simulink model "all_afc_0001_0365"  (R2026a)
settings: Solver=ode15s  StopTime=simTime  FixedStep=5e-05  RelTol=1e-06  AbsTol=1e-06
undefined symbols (not defined in the file): AF_sensor_tol, fault_time, fuel_inj_tol, MAF_sensor_tol, measureTime, simTime, spec_num
(part 2 of 3)

== system all_afc_0001_0365/Model 1/Cylinder and Exhaust/A//F_sensor ==
  In : Inport
  A/F_sensor : Gain  OutDataTypeStr=double
  FIMWB_133 : Subsystem  Tag=fimwb.fault.133
  FIMWB_134 : Subsystem  Tag=fimwb.fault.134
  FIMWB_135 : Subsystem  Tag=fimwb.fault.135
  Filter : Subsystem
  Out : Outport  VectorParamsAs1DForOutWhenUnconnected=off
  wires:
  In/1 -> FIMWB_133/1(Original)
  FIMWB_133/1(Result) -> Filter/1(In)
  A/F_sensor/1 -> FIMWB_134/1(Original)
  FIMWB_134/1(Result) -> Out/1
  Filter/1(Out) -> FIMWB_135/1(Original)
  FIMWB_135/1(Result) -> A/F_sensor/1

== system all_afc_0001_0365/Model 1/Cylinder and Exhaust/FIMWB_125 ==
  Original : Inport
  Result : Outport
  wires:
  Original/1 -> Result/1

== system all_afc_0001_0365/Model 1/Cylinder and Exhaust/FIMWB_126 ==
  Original : Inport
  Result : Outport
  wires:
  Original/1 -> Result/1

== system all_afc_0001_0365/Model 1/Cylinder and Exhaust/FIMWB_127 ==
  Original : Inport
  Result : Outport
  wires:
  Original/1 -> Result/1

== system all_afc_0001_0365/Model 1/Cylinder and Exhaust/FIMWB_128 ==
  Original : Inport
  Result : Outport
  wires:
  Original/1 -> Result/1

== system all_afc_0001_0365/Model 1/Cylinder and Exhaust/FIMWB_129 ==
  Original : Inport
  Result : Outport
  wires:
  Original/1 -> Result/1

== system all_afc_0001_0365/Model 1/Cylinder and Exhaust/FIMWB_130 ==
  Original : Inport
  Result : Outport
  wires:
  Original/1 -> Result/1

== system all_afc_0001_0365/Model 1/Cylinder and Exhaust/FIMWB_131 ==
  Original : Inport
  Result : Outport
  wires:
  Original/1 -> Result/1

== system all_afc_0001_0365/Model 1/Cylinder and Exhaust/FIMWB_132 ==
  Original : Inport
  Result : Outport
  wires:
  Original/1 -> Result/1

== system all_afc_0001_0365/Model 1/Cylinder and Exhaust/FIMWB_141 ==
  Original : Inport
  Result : Outport
  wires:
  Original/1 -> Result/1

== system all_afc_0001_0365/Model 1/Cylinder and Exhaust/FIMWB_142 ==
  Original : Inport
  Result : Outport
  wires:
  Original/1 -> Result/1

== system all_afc_0001_0365/Model 1/Cylinder and Exhaust/FIMWB_143 ==
  Original : Inport
  Result : Outport
  wires:
  Original/1 -> Result/1

== system all_afc_0001_0365/Model 1/Cylinder and Exhaust/FIMWB_149 ==
  Original : Inport
  Result : Outport
  wires:
  Original/1 -> Result/1

== system all_afc_0001_0365/Model 1/Cylinder and Exhaust/FIMWB_150 ==
  Original : Inport
  Result : Outport
  wires:
  Original/1 -> Result/1

== system all_afc_0001_0365/Model 1/Cylinder and Exhaust/FIMWB_151 ==
  Original : Inport
  Result : Outport
  wires:
  Original/1 -> Result/1

== system all_afc_0001_0365/Model 1/Cylinder and Exhaust/FIMWB_152 ==
  Original : Inport
  Result : Outport
  wires:
  Original/1 -> Result/1

== system all_afc_0001_0365/Model 1/Cylinder and Exhaust/FIMWB_153 ==
  Original : Inport
  Result : Outport
  wires:
  Original/1 -> Result/1

== system all_afc_0001_0365/Model 1/Cylinder and Exhaust/FIMWB_154 ==
  Original : Inport
  Result : Outport
  wires:
  Original/1 -> Result/1

== system all_afc_0001_0365/Model 1/Cylinder and Exhaust/FIMWB_155 ==
  Original : Inport
  Result : Outport
  wires:
  Original/1 -> Result/1

== system all_afc_0001_0365/Model 1/Cylinder and Exhaust/FIMWB_156 ==
  Original : Inport
  Result : Outport
  wires:
  Original/1 -> Result/1

== system all_afc_0001_0365/Model 1/Cylinder and Exhaust/FIMWB_157 ==
  Original : Inport
  Result : Outport
  wires:
  Original/1 -> Result/1

== system all_afc_0001_0365/Model 1/Cylinder and Exhaust/FIMWB_304 ==
  Original : Inport
  Operand1 : Inport  Port=2
  Operand2 : Inport  Port=3
  Unused2 : Terminator
  Unused3 : Terminator
  Result : Outport
  wires:
  Original/1 -> Result/1
  Operand1/1 -> Unused2/1
  Operand2/1 -> Unused3/1

== system all_afc_0001_0365/Model 1/Cylinder and Exhaust/FIMWB_306 ==
  Original : Inport
  Operand1 : Inport  Port=2
  Operand2 : Inport  Port=3
  Unused2 : Terminator
  Unused3 : Terminator
  Result : Outport
  wires:
  Original/1 -> Result/1
  Operand1/1 -> Unused2/1
  Operand2/1 -> Unused3/1

== system all_afc_0001_0365/Model 1/Cylinder and Exhaust/FIMWB_342 ==
  Original : Inport
  Result : Outport
  wires:
  Original/1 -> Result/1

== system all_afc_0001_0365/Model 1/Cylinder and Exhaust/FIMWB_343 ==
  Original : Inport
  Result : Outport
  wires:
  Original/1 -> Result/1

== system all_afc_0001_0365/Model 1/Cylinder and Exhaust/FIMWB_344 ==
  Original : Inport
  Result : Outport
  wires:
  Original/1 -> Result/1

== system all_afc_0001_0365/Model 1/Cylinder and Exhaust/FIMWB_347 ==
  Original : Inport
  Result : Outport
  wires:
  Original/1 -> Result/1

== system all_afc_0001_0365/Model 1/Cylinder and Exhaust/Filter ==
  in : Inport
  FIMWB_144 : Subsystem  Tag=fimwb.fault.144
  FIMWB_145 : Subsystem  Tag=fimwb.fault.145
  FIMWB_146 : Subsystem  Tag=fimwb.fault.146
  FIMWB_147 : Subsystem  Tag=fimwb.fault.147
  FIMWB_148 : Subsystem  Tag=fimwb.fault.148
  FIMWB_305 : Subsystem  Tag=fimwb.fault.305
  FIMWB_346 : Subsystem  Tag=fimwb.fault.346
  Gain1 : Gain  Gain=10
  Integrator : Integrator  InitialCondition=14.7
  Sum : Sum  Inputs=|+-
  out : Outport  VectorParamsAs1DForOutWhenUnconnected=off
  wires:
  Sum/1 -> FIMWB_305/1(Original)
  Integrator/1 -> FIMWB_346/1(Original)
  FIMWB_346/1(Result) -> FIMWB_146/1(Original), FIMWB_147/1(Original)
  in/1 -> FIMWB_144/1(Original)
  FIMWB_144/1(Result) -> Sum/1, FIMWB_305/2(Operand1)
  Gain1/1 -> FIMWB_145/1(Original)
  FIMWB_145/1(Result) -> Integrator/1
  FIMWB_146/1(Result) -> Sum/2, FIMWB_305/3(Operand2)
  FIMWB_147/1(Result) -> out/1
  FIMWB_305/1(Result) -> FIMWB_148/1(Original)
  FIMWB_148/1(Result) -> Gain1/1

== system all_afc_0001_0365/Model 1/Intake Manifold/FIMWB_174 ==
  Original : Inport
  Result : Outport
  wires:
  Original/1 -> Result/1

== system all_afc_0001_0365/Model 1/Intake Manifold/FIMWB_175 ==
  Original : Inport
  Result : Outport
  wires:
  Original/1 -> Result/1

== system all_afc_0001_0365/Model 1/Intake Manifold/FIMWB_176 ==
  Original : Inport
  Result : Outport
  wires:
  Original/1 -> Result/1

== system all_afc_0001_0365/Model 1/Intake Manifold/FIMWB_177 ==
  Original : Inport
  Result : Outport
  wires:
  Original/1 -> Result/1

== system all_afc_0001_0365/Model 1/Intake Manifold/FIMWB_178 ==
  Original : Inport
  Result : Outport
  wires:
  Original/1 -> Result/1

== system all_afc_0001_0365/Model 1/Intake Manifold/FIMWB_179 ==
  Original : Inport
  Result : Outport
  wires:
  Original/1 -> Result/1

== system all_afc_0001_0365/Model 1/Intake Manifold/FIMWB_180 ==
  Original : Inport
  Result : Outport
  wires:
  Original/1 -> Result/1

== system all_afc_0001_0365/Model 1/Intake Manifold/FIMWB_181 ==
  Original : Inport
  Result : Outport
  wires:
  Original/1 -> Result/1

== system all_afc_0001_0365/Model 1/Intake Manifold/FIMWB_182 ==
  Original : Inport
  Result : Outport
  wires:
  Original/1 -> Result/1

== system all_afc_0001_0365/Model 1/Intake Manifold/FIMWB_183 ==
  Original : Inport
  Result : Outport
  wires:
  Original/1 -> Result/1

== system all_afc_0001_0365/Model 1/Intake Manifold/FIMWB_307 ==
  Original : Inport
  Operand1 : Inport  Port=2
  Operand2 : Inport  Port=3
  Unused2 : Terminator
  Unused3 : Terminator
  Result : Outport
  wires:
  Original/1 -> Result/1
  Operand1/1 -> Unused2/1
  Operand2/1 -> Unused3/1

== system all_afc_0001_0365/Model 1/Intake Manifold/FIMWB_348 ==
  Original : Inport
  Result : Outport
  wires:
  Original/1 -> Result/1

== system all_afc_0001_0365/Model 1/Intake Manifold/FIMWB_349 ==
  Original : Inport
  Result : Outport
  wires:
  Original/1 -> Result/1

== system all_afc_0001_0365/Model 1/Throttle/FIMWB_188 ==
  Original : Inport
  Result : Outport
  wires:
  Original/1 -> Result/1

== system all_afc_0001_0365/Model 1/Throttle/FIMWB_189 ==
  Original : Inport
  Result : Outport
  wires:
  Original/1 -> Result/1

== system all_afc_0001_0365/Model 1/Throttle/FIMWB_190 ==
  Original : Inport
  Result : Outport
  wires:
  Original/1 -> Result/1

== system all_afc_0001_0365/Model 1/Throttle/FIMWB_191 ==
  Original : Inport
  Result : Outport
  wires:
  Original/1 -> Result/1

== system all_afc_0001_0365/Model 1/Throttle/FIMWB_192 ==
  Original : Inport
  Result : Outport
  wires:
  Original/1 -> Result/1

== system all_afc_0001_0365/Model 1/Throttle/FIMWB_193 ==
  Original : Inport
  Result : Outport
  wires:
  Original/1 -> Result/1

== system all_afc_0001_0365/Model 1/Throttle/FIMWB_194 ==
  Original : Inport
  Result : Outport
  wires:
  Original/1 -> Result/1

== system all_afc_0001_0365/Model 1/Throttle/FIMWB_195 ==
  Original : Inport
  Result : Outport
  wires:
  Original/1 -> Result/1

== system all_afc_0001_0365/Model 1/Throttle/FIMWB_196 ==
  Original : Inport
  Result : Outport
  wires:
  Original/1 -> Result/1

== system all_afc_0001_0365/Model 1/Throttle/FIMWB_197 ==
  Original : Inport
  Result : Outport
  wires:
  Original/1 -> Result/1

== system all_afc_0001_0365/Model 1/Throttle/FIMWB_198 ==
  Original : Inport
  Result : Outport
  wires:
  Original/1 -> Result/1

== system all_afc_0001_0365/Model 1/Throttle/FIMWB_199 ==
  Original : Inport
  Result : Outport
  wires:
  Original/1 -> Result/1

== system all_afc_0001_0365/Model 1/Throttle/FIMWB_200 ==
  Original : Inport
  Result : Outport
  wires:
  Original/1 -> Result/1

== system all_afc_0001_0365/Model 1/Throttle/FIMWB_201 ==
  Original : Inport
  Result : Outport
  wires:
  Original/1 -> Result/1

== system all_afc_0001_0365/Model 1/Throttle/FIMWB_202 ==
  Original : Inport
  Result : Outport
  wires:
  Original/1 -> Result/1

== system all_afc_0001_0365/Model 1/Throttle/FIMWB_203 ==
  Original : Inport
  Result : Outport
  wires:
  Original/1 -> Result/1

== system all_afc_0001_0365/Model 1/Throttle/FIMWB_204 ==
  Original : Inport
  Result : Outport
  wires:
  Original/1 -> Result/1

== system all_afc_0001_0365/Model 1/Throttle/FIMWB_205 ==
  Original : Inport
  Result : Outport
  wires:
  Original/1 -> Result/1

== system all_afc_0001_0365/Model 1/Throttle/FIMWB_309 ==
  Original : Inport
  Operand1 : Inport  Port=2
  Operand2 : Inport  Port=3
  Operand3 : Inport  Port=4
  Unused2 : Terminator
  Unused3 : Terminator
  Unused4 : Terminator
  Result : Outport
  wires:
  Original/1 -> Result/1
  Operand1/1 -> Unused2/1
  Operand2/1 -> Unused3/1
  Operand3/1 -> Unused4/1

== system all_afc_0001_0365/Model 1/Throttle/FIMWB_310 ==
  Original : Inport
  Operand1 : Inport  Port=2
  Operand2 : Inport  Port=3
  Unused2 : Terminator
  Unused3 : Terminator
  Result : Outport
  wires:
  Original/1 -> Result/1
  Operand1/1 -> Unused2/1
  Operand2/1 -> Unused3/1

== system all_afc_0001_0365/Model 1/Throttle/FIMWB_311 ==
  Original : Inport
  Operand1 : Inport  Port=2
  Operand2 : Inport  Port=3
  Unused2 : Terminator
  Unused3 : Terminator
  Result : Outport
  wires:
  Original/1 -> Result/1
  Operand1/1 -> Unused2/1
  Operand2/1 -> Unused3/1

== system all_afc_0001_0365/Model 1/Throttle/FIMWB_312 ==
  Original : Inport
  Operand1 : Inport  Port=2
  Operand2 : Inport  Port=3
  Unused2 : Terminator
  Unused3 : Terminator
  Result : Outport
  wires:
  Original/1 -> Result/1
  Operand1/1 -> Unused2/1
  Operand2/1 -> Unused3/1

== system all_afc_0001_0365/Model 1/Throttle/FIMWB_351 ==
  Original : Inport
  Result : Outport
  wires:
  Original/1 -> Result/1

== system all_afc_0001_0365/Model 1/Throttle/FIMWB_352 ==
  Original : Inport
  Result : Outport
  wires:
  Original/1 -> Result/1

== system all_afc_0001_0365/Model 1/Throttle/FIMWB_353 ==
  Original : Inport
  Result : Outport
  wires:
  Original/1 -> Result/1

== system all_afc_0001_0365/Model 1/Wall wetting/FIMWB_208 ==
  Original : Inport
  Result : Outport
  wires:
  Original/1 -> Result/1

== system all_afc_0001_0365/Model 1/Wall wetting/FIMWB_209 ==
  Original : Inport
  Result : Outport
  wires:
  Original/1 -> Result/1

== system all_afc_0001_0365/Model 1/Wall wetting/FIMWB_210 ==
  Original : Inport
  Result : Outport
  wires:
  Original/1 -> Result/1

== system all_afc_0001_0365/Model 1/Wall wetting/FIMWB_211 ==
  Original : Inport
  Result : Outport
  wires:
  Original/1 -> Result/1

== system all_afc_0001_0365/Model 1/Wall wetting/FIMWB_212 ==
  Original : Inport
  Result : Outport
  wires:
  Original/1 -> Result/1

== system all_afc_0001_0365/Model 1/Wall wetting/FIMWB_213 ==
  Original : Inport
  Result : Outport
  wires:
  Original/1 -> Result/1

== system all_afc_0001_0365/Model 1/Wall wetting/FIMWB_214 ==
  Original : Inport
  Result : Outport
  wires:
  Original/1 -> Result/1

== system all_afc_0001_0365/Model 1/Wall wetting/FIMWB_215 ==
  Original : Inport
  Result : Outport
  wires:
  Original/1 -> Result/1

== system all_afc_0001_0365/Model 1/Wall wetting/FIMWB_216 ==
  Original : Inport
  Result : Outport
  wires:
  Original/1 -> Result/1

== system all_afc_0001_0365/Model 1/Wall wetting/FIMWB_217 ==
  Original : Inport
  Result : Outport
  wires:
  Original/1 -> Result/1

== system all_afc_0001_0365/Model 1/Wall wetting/FIMWB_218 ==
  Original : Inport
  Result : Outport
  wires:
  Original/1 -> Result/1

== system all_afc_0001_0365/Model 1/Wall wetting/FIMWB_219 ==
  Original : Inport
  Result : Outport
  wires:
  Original/1 -> Result/1

== system all_afc_0001_0365/Model 1/Wall wetting/FIMWB_220 ==
  Original : Inport
  Result : Outport
  wires:
  Original/1 -> Result/1

== system all_afc_0001_0365/Model 1/Wall wetting/FIMWB_221 ==
  Original : Inport
  Result : Outport
  wires:
  Original/1 -> Result/1

== system all_afc_0001_0365/Model 1/Wall wetting/FIMWB_222 ==
  Original : Inport
  Result : Outport
  wires:
  Original/1 -> Result/1

== system all_afc_0001_0365/Model 1/Wall wetting/FIMWB_223 ==
  Original : Inport
  Result : Outport
  wires:
  Original/1 -> Result/1

== system all_afc_0001_0365/Model 1/Wall wetting/FIMWB_224 ==
  Original : Inport
  Result : Outport
  wires:
  Original/1 -> Result/1

== system all_afc_0001_0365/Model 1/Wall wetting/FIMWB_225 ==
  Original : Inport
  Result : Outport
  wires:
  Original/1 -> Result/1

== system all_afc_0001_0365/Model 1/Wall wetting/FIMWB_226 ==
  Original : Inport
  Result : Outport
  wires:
  Original/1 -> Result/1

== system all_afc_0001_0365/Model 1/Wall wetting/FIMWB_227 ==
  Original : Inport
  Result : Outport
  wires:
  Original/1 -> Result/1

== system all_afc_0001_0365/Model 1/Wall wetting/FIMWB_228 ==
  Original : Inport
  Result : Outport
  wires:
  Original/1 -> Result/1

== system all_afc_0001_0365/Model 1/Wall wetting/FIMWB_229 ==
  Original : Inport
  Result : Outport
  wires:
  Original/1 -> Result/1

== system all_afc_0001_0365/Model 1/Wall wetting/FIMWB_230 ==
  Original : Inport
  Result : Outport
  wires:
  Original/1 -> Result/1

== system all_afc_0001_0365/Model 1/Wall wetting/FIMWB_231 ==
  Original : Inport
  Result : Outport
  wires:
  Original/1 -> Result/1

== system all_afc_0001_0365/Model 1/Wall wetting/FIMWB_313 ==
  Original : Inport
  Operand1 : Inport  Port=2
  Operand2 : Inport  Port=3
  Unused2 : Terminator
  Unused3 : Terminator
  Result : Outport
  wires:
  Original/1 -> Result/1
  Operand1/1 -> Unused2/1
  Operand2/1 -> Unused3/1

== system all_afc_0001_0365/Model 1/Wall wetting/FIMWB_314 ==
  Original : Inport
  Operand1 : Inport  Port=2
  Operand2 : Inport  Port=3
  Unused2 : Terminator
  Unused3 : Terminator
  Result : Outport
  wires:
  Original/1 -> Result/1
  Operand1/1 -> Unused2/1
  Operand2/1 -> Unused3/1

== system all_afc_0001_0365/Model 1/Wall wetting/FIMWB_315 ==
  Original : Inport
  Operand1 : Inport  Port=2
  Operand2 : Inport  Port=3
  Unused2 : Terminator
  Unused3 : Terminator
  Result : Outport
  wires:
  Original/1 -> Result/1
  Operand1/1 -> Unused2/1
  Operand2/1 -> Unused3/1

== system all_afc_0001_0365/Model 1/Wall wetting/FIMWB_316 ==
  Original : Inport
  Operand1 : Inport  Port=2
  Operand2 : Inport  Port=3
  Unused2 : Terminator
  Unused3 : Terminator
  Result : Outport
  wires:
  Original/1 -> Result/1
  Operand1/1 -> Unused2/1
  Operand2/1 -> Unused3/1

== system all_afc_0001_0365/Model 1/Wall wetting/FIMWB_317 ==
  Original : Inport
  Operand1 : Inport  Port=2
  Operand2 : Inport  Port=3
  Unused2 : Terminator
  Unused3 : Terminator
  Result : Outport
  wires:
  Original/1 -> Result/1
  Operand1/1 -> Unused2/1
  Operand2/1 -> Unused3/1

== system all_afc_0001_0365/Model 1/Wall wetting/FIMWB_318 ==
  Original : Inport
  Operand1 : Inport  Port=2
  Operand2 : Inport  Port=3
  Unused2 : Terminator
  Unused3 : Terminator
  Result : Outport
  wires:
  Original/1 -> Result/1
  Operand1/1 -> Unused2/1
  Operand2/1 -> Unused3/1

== system all_afc_0001_0365/Model 1/Wall wetting/FIMWB_354 ==
  Original : Inport
  Result : Outport
  wires:
  Original/1 -> Result/1

== system all_afc_0001_0365/Model 1/Wall wetting/FIMWB_355 ==
  Original : Inport
  Result : Outport
  wires:
  Original/1 -> Result/1

== system all_afc_0001_0365/Model 1/Wall wetting/FIMWB_356 ==
  Original : Inport
  Result : Outport
  wires:
  Original/1 -> Result/1

== system all_afc_0001_0365/Model 1/Wall wetting/FIMWB_357 ==
  Original : Inport
  Result : Outport
  wires:
  Original/1 -> Result/1

== system all_afc_0001_0365/Model 1/Wall wetting/FIMWB_358 ==
  Original : Inport
  Result : Outport
  wires:
  Original/1 -> Result/1

== system all_afc_0001_0365/V&V stub system/Calcuate Error/FIMWB_241 ==
  Original : Inport
  Result : Outport
  wires:
  Original/1 -> Result/1

== system all_afc_0001_0365/V&V stub system/Calcuate Error/FIMWB_242 ==
  Original : Inport
  Result : Outport
  wires:
  Original/1 -> Result/1

== system all_afc_0001_0365/V&V stub system/Calcuate Error/FIMWB_243 ==
  Original : Inport
  Result : Outport
  wires:
  Original/1 -> Result/1

== system all_afc_0001_0365/V&V stub system/Calcuate Error/FIMWB_244 ==
  Original : Inport
  Result : Outport
  wires:
  Original/1 -> Result/1

== system all_afc_0001_0365/V&V stub system/Calcuate Error/FIMWB_245 ==
  Original : Inport
  Result : Outport
  wires:
  Original/1 -> Result/1

== system all_afc_0001_0365/V&V stub system/Calcuate Error/FIMWB_246 ==
  Original : Inport
  Result : Outport
  wires:
  Original/1 -> Result/1

== system all_afc_0001_0365/V&V stub system/Calcuate Error/FIMWB_247 ==
  Original : Inport
  Result : Outport
  wires:
  Original/1 -> Result/1

== system all_afc_0001_0365/V&V stub system/Calcuate Error/FIMWB_255 ==
  Original : Inport
  Result : Outport
  wires:
  Original/1 -> Result/1

== system all_afc_0001_0365/V&V stub system/Calcuate Error/FIMWB_272 ==
  Original : Inport
  Result : Outport
  wires:
  Original/1 -> Result/1

== system all_afc_0001_0365/V&V stub system/Calcuate Error/FIMWB_273 ==
  Original : Inport
  Result : Outport
  wires:
  Original/1 -> Result/1

== system all_afc_0001_0365/V&V stub system/Calcuate Error/FIMWB_274 ==
  Original : Inport
  Result : Outport
  wires:
  Original/1 -> Result/1

== system all_afc_0001_0365/V&V stub system/Calcuate Error/FIMWB_362 ==
  Original : Inport
  Result : Outport
  wires:
  Original/1 -> Result/1

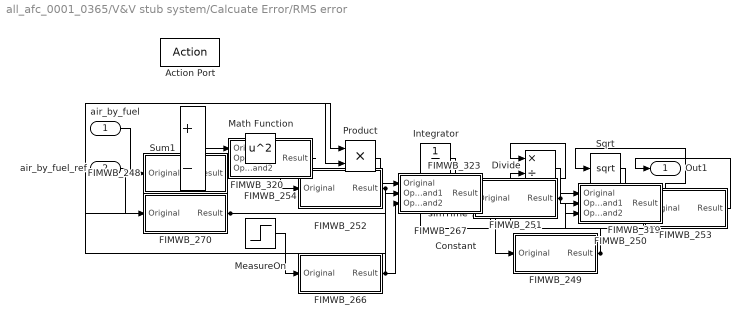
== system all_afc_0001_0365/V&V stub system/Calcuate Error/RMS error ==
  "air_by_fuel " : Inport
  air_by_fuel_ref : Inport  Port=2
  Action Port : ActionPort  ActionPortLabel=case: { }
  Constant : Constant  Value=simTime-10
  Divide : Product  Inputs=*/
  FIMWB_248 : Subsystem  Tag=fimwb.fault.248
  FIMWB_249 : Subsystem  Tag=fimwb.fault.249
  FIMWB_250 : Subsystem  Tag=fimwb.fault.250
  FIMWB_251 : Subsystem  Tag=fimwb.fault.251
  FIMWB_252 : Subsystem  Tag=fimwb.fault.252
  FIMWB_253 : Subsystem  Tag=fimwb.fault.253
  FIMWB_254 : Subsystem  Tag=fimwb.fault.254
  FIMWB_266 : Subsystem  Tag=fimwb.fault.266
  FIMWB_267 : Subsystem  Tag=fimwb.fault.267
  FIMWB_270 : Subsystem  Tag=fimwb.fault.270
  FIMWB_319 : Subsystem  Tag=fimwb.fault.319
  FIMWB_320 : Subsystem  Tag=fimwb.fault.320
  FIMWB_323 : Subsystem  Tag=fimwb.fault.323
  Integrator : Integrator
  Math Function : Math  Operator=square  SignedPower=on
  MeasureOn : Step  Time=10  SampleTime=0
  Product : Product
  Sqrt : Sqrt
  Sum1 : Sum  Inputs=+-  OutDataTypeStr=Inherit: Inherit via back propagation  InputSameDT=on  RndMeth=Simplest
  Out1 : Outport  VectorParamsAs1DForOutWhenUnconnected=off
  wires:
  Divide/1 -> FIMWB_319/1(Original)
  Sum1/1 -> FIMWB_320/1(Original)
  Product/1 -> FIMWB_323/1(Original)
  "air_by_fuel "/1 -> FIMWB_248/1(Original)
  FIMWB_248/1(Result) -> Sum1/1, FIMWB_320/2(Operand1)
  Constant/1 -> FIMWB_249/1(Original)
  FIMWB_249/1(Result) -> Divide/2, FIMWB_319/3(Operand2)
  FIMWB_319/1(Result) -> FIMWB_250/1(Original)
  FIMWB_250/1(Result) -> Sqrt/1
  Integrator/1 -> FIMWB_251/1(Original)
  FIMWB_251/1(Result) -> Divide/1, FIMWB_319/2(Operand1)
  Math Function/1 -> FIMWB_252/1(Original)
  FIMWB_252/1(Result) -> Product/1, FIMWB_323/2(Operand1)
  Sqrt/1 -> FIMWB_253/1(Original)
  FIMWB_253/1(Result) -> Out1/1
  FIMWB_320/1(Result) -> FIMWB_254/1(Original)
  FIMWB_254/1(Result) -> Math Function/1
  MeasureOn/1 -> FIMWB_266/1(Original)
  FIMWB_266/1(Result) -> Product/2, FIMWB_323/3(Operand2)
  FIMWB_323/1(Result) -> FIMWB_267/1(Original)
  FIMWB_267/1(Result) -> Integrator/1
  air_by_fuel_ref/1 -> FIMWB_270/1(Original)
  FIMWB_270/1(Result) -> Sum1/2, FIMWB_320/3(Operand2)

== system all_afc_0001_0365/V&V stub system/Calcuate Error/over(under)shoot ==
  "air_by_fuel " : Inport
  air_by_fuel_ref : Inport  Port=2
  Action Port : ActionPort  ActionPortLabel=case: { }
  Constant : Constant
  Divide : Product  Inputs=*/
  FIMWB_256 : Subsystem  Tag=fimwb.fault.256
  FIMWB_257 : Subsystem  Tag=fimwb.fault.257
  FIMWB_258 : Subsystem  Tag=fimwb.fault.258
  FIMWB_259 : Subsystem  Tag=fimwb.fault.259
  FIMWB_271 : Subsystem  Tag=fimwb.fault.271
  FIMWB_321 : Subsystem  Tag=fimwb.fault.321
  FIMWB_322 : Subsystem  Tag=fimwb.fault.322
  Sum1 : Sum  Inputs=+-  OutDataTypeStr=Inherit: Inherit via back propagation  InputSameDT=on  RndMeth=Simplest
  Out1 : Outport  VectorParamsAs1DForOutWhenUnconnected=off
  wires:
  Divide/1 -> FIMWB_321/1(Original)
  Sum1/1 -> FIMWB_322/1(Original)
  "air_by_fuel "/1 -> FIMWB_256/1(Original)
  FIMWB_256/1(Result) -> Divide/1, FIMWB_321/2(Operand1)
  Constant/1 -> FIMWB_257/1(Original)
  FIMWB_257/1(Result) -> Sum1/2, FIMWB_322/3(Operand2)
  FIMWB_321/1(Result) -> FIMWB_258/1(Original)
  FIMWB_258/1(Result) -> Sum1/1, FIMWB_322/2(Operand1)
  FIMWB_322/1(Result) -> FIMWB_259/1(Original)
  FIMWB_259/1(Result) -> Out1/1
  air_by_fuel_ref/1 -> FIMWB_271/1(Original)
  FIMWB_271/1(Result) -> Divide/2, FIMWB_321/3(Operand2)

== system all_afc_0001_0365/Model 1/AF_Controller/fuel_controller/FIMWB_021 ==
  Original : Inport
  Result : Outport
  wires:
  Original/1 -> Result/1

== system all_afc_0001_0365/Model 1/AF_Controller/fuel_controller/FIMWB_022 ==
  Original : Inport
  Result : Outport
  wires:
  Original/1 -> Result/1

== system all_afc_0001_0365/Model 1/AF_Controller/fuel_controller/FIMWB_023 ==
  Original : Inport
  Result : Outport
  wires:
  Original/1 -> Result/1

== system all_afc_0001_0365/Model 1/AF_Controller/fuel_controller/FIMWB_024 ==
  Original : Inport
  Result : Outport
  wires:
  Original/1 -> Result/1

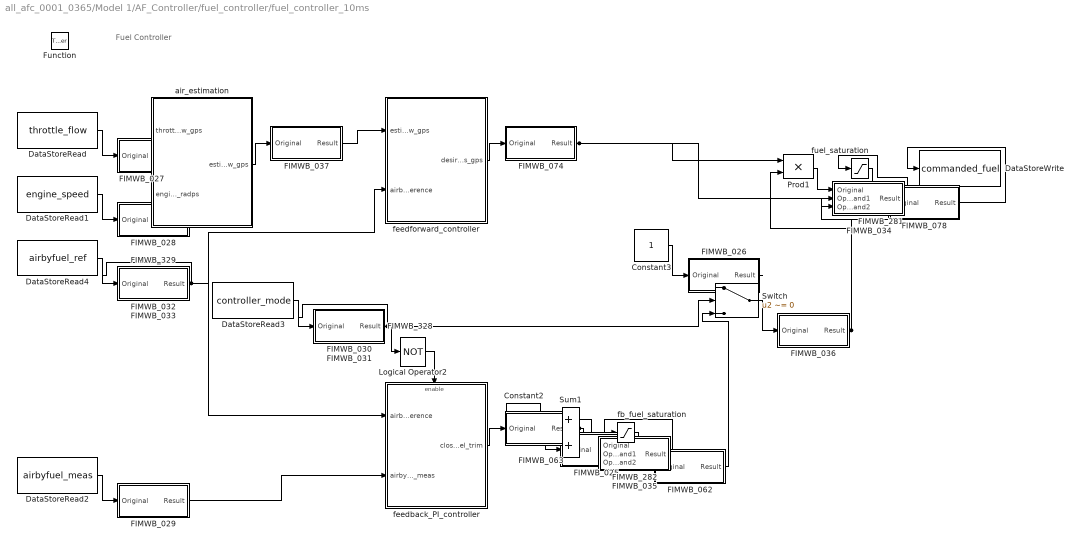
== system all_afc_0001_0365/Model 1/AF_Controller/fuel_controller/fuel_controller_10ms ==
  note: Fuel Controller
  Function : TriggerPort  VariantControl=(inherit)
  Constant2 : Constant  OutDataTypeStr=single
  Constant3 : Constant  OutDataTypeStr=single
  DataStoreRead : DataStoreRead  DataStoreName=throttle_flow  IndexOptions=Index vector (dialog)  Indices=1  OutputSizes=1
  DataStoreRead1 : DataStoreRead  DataStoreName=engine_speed  IndexOptions=Index vector (dialog)  Indices=1  OutputSizes=1
  DataStoreRead2 : DataStoreRead  DataStoreName=airbyfuel_meas  IndexOptions=Index vector (dialog)  Indices=1  OutputSizes=1
  DataStoreRead3 : DataStoreRead  DataStoreName=controller_mode  IndexOptions=Index vector (dialog)  Indices=1  OutputSizes=1
      settings: AttributesFormatString=1: Feedforward\n0: Feedforward + Feedback
  DataStoreRead4 : DataStoreRead  DataStoreName=airbyfuel_ref  IndexOptions=Index vector (dialog)  Indices=1  OutputSizes=1
  DataStoreWrite : DataStoreWrite  DataStoreName=commanded_fuel  IndexOptions=Index vector (dialog)  Indices=1  OutputSizes=1
  FIMWB_025 : Subsystem  Tag=fimwb.fault.25
  FIMWB_026 : Subsystem  Tag=fimwb.fault.26
  FIMWB_027 : Subsystem  Tag=fimwb.fault.27
  FIMWB_028 : Subsystem  Tag=fimwb.fault.28
  FIMWB_029 : Subsystem  Tag=fimwb.fault.29
  FIMWB_030 : Subsystem  Tag=fimwb.fault.30
  FIMWB_031 : Subsystem  Tag=fimwb.fault.31
  FIMWB_032 : Subsystem  Tag=fimwb.fault.32
  FIMWB_033 : Subsystem  Tag=fimwb.fault.33
  FIMWB_034 : Subsystem  Tag=fimwb.fault.34
  FIMWB_035 : Subsystem  Tag=fimwb.fault.35
  FIMWB_036 : Subsystem  Tag=fimwb.fault.36
  FIMWB_037 : Subsystem  Tag=fimwb.fault.37
  FIMWB_062 : Subsystem  Tag=fimwb.fault.62
  FIMWB_063 : Subsystem  Tag=fimwb.fault.63
  FIMWB_074 : Subsystem  Tag=fimwb.fault.74
  FIMWB_078 : Subsystem  Tag=fimwb.fault.78
  FIMWB_281 : Subsystem  Tag=fimwb.fault.281
  FIMWB_282 : Subsystem  Tag=fimwb.fault.282
  FIMWB_328 : Subsystem  Tag=fimwb.fault.328
  FIMWB_329 : Subsystem  Tag=fimwb.fault.329
  Logical Operator2 : Logic  Operator=NOT  AllPortsSameDT=off  OutDataTypeStr=boolean
  Prod1 : Product  OutDataTypeStr=Inherit: Inherit via back propagation  RndMeth=Simplest
  Sum1 : Sum  OutDataTypeStr=Inherit: Inherit via back propagation  InputSameDT=on  RndMeth=Simplest
  Switch : Switch  Criteria=u2 ~= 0  Threshold=0.5  SaturateOnIntegerOverflow=off  InputSameDT=off
  air_estimation : Subsystem  TreatAsAtomicUnit=on
  fb_fuel_saturation : Saturate  UpperLimit=inf  LowerLimit=0  RndMeth=Round
      settings: AttributesFormatString=y >= 0
  feedback_PI_controller : Subsystem  TreatAsAtomicUnit=on
  feedforward_controller : Subsystem  TreatAsAtomicUnit=on
  fuel_saturation : Saturate  UpperLimit=1.66  LowerLimit=0.13  RndMeth=Round
      settings: AttributesFormatString=0.13 <=\ncommanded_fuel\n<= 1.66
  wires:
  Logical Operator2/1 -> feedback_PI_controller/Enable
  Prod1/1 -> FIMWB_281/1(Original)
  Sum1/1 -> FIMWB_282/1(Original)
  DataStoreRead3/1 -> FIMWB_328/1(Original)
  FIMWB_328/1(Result) -> FIMWB_030/1(Original), FIMWB_031/1(Original)
  DataStoreRead4/1 -> FIMWB_329/1(Original)
  FIMWB_329/1(Result) -> FIMWB_032/1(Original), FIMWB_033/1(Original)
  Constant2/1 -> FIMWB_025/1(Original)
  FIMWB_025/1(Result) -> Sum1/1, FIMWB_282/2(Operand1)
  Constant3/1 -> FIMWB_026/1(Original)
  FIMWB_026/1(Result) -> Switch/1
  DataStoreRead/1 -> FIMWB_027/1(Original)
  FIMWB_027/1(Result) -> air_estimation/1(throttle_flow_gps)
  DataStoreRead1/1 -> FIMWB_028/1(Original)
  FIMWB_028/1(Result) -> air_estimation/2(engine_speed_radps)
  DataStoreRead2/1 -> FIMWB_029/1(Original)
  FIMWB_029/1(Result) -> feedback_PI_controller/2(airbyfuel_meas)
  FIMWB_030/1(Result) -> Logical Operator2/1
  FIMWB_031/1(Result) -> Switch/2
  FIMWB_032/1(Result) -> feedback_PI_controller/1(airbyfuel_reference)
  FIMWB_033/1(Result) -> feedforward_controller/2(airbyfuel_reference)
  FIMWB_281/1(Result) -> FIMWB_034/1(Original)
  FIMWB_034/1(Result) -> fuel_saturation/1
  FIMWB_282/1(Result) -> FIMWB_035/1(Original)
  FIMWB_035/1(Result) -> fb_fuel_saturation/1
  Switch/1 -> FIMWB_036/1(Original)
  FIMWB_036/1(Result) -> Prod1/2, FIMWB_281/3(Operand2)
  air_estimation/1(estimated_cyl_air_flow_gps) -> FIMWB_037/1(Original)
  FIMWB_037/1(Result) -> feedforward_controller/1(estimated_cyl_air_flow_gps)
  fb_fuel_saturation/1 -> FIMWB_062/1(Original)
  FIMWB_062/1(Result) -> Switch/3
  feedback_PI_controller/1(closed_loop_fuel_trim) -> FIMWB_063/1(Original)
  FIMWB_063/1(Result) -> Sum1/2, FIMWB_282/3(Operand2)
  feedforward_controller/1(desired_fuel_mass_gps) -> FIMWB_074/1(Original)
  FIMWB_074/1(Result) -> Prod1/1, FIMWB_281/2(Operand1)
  fuel_saturation/1 -> FIMWB_078/1(Original)
  FIMWB_078/1(Result) -> DataStoreWrite/1

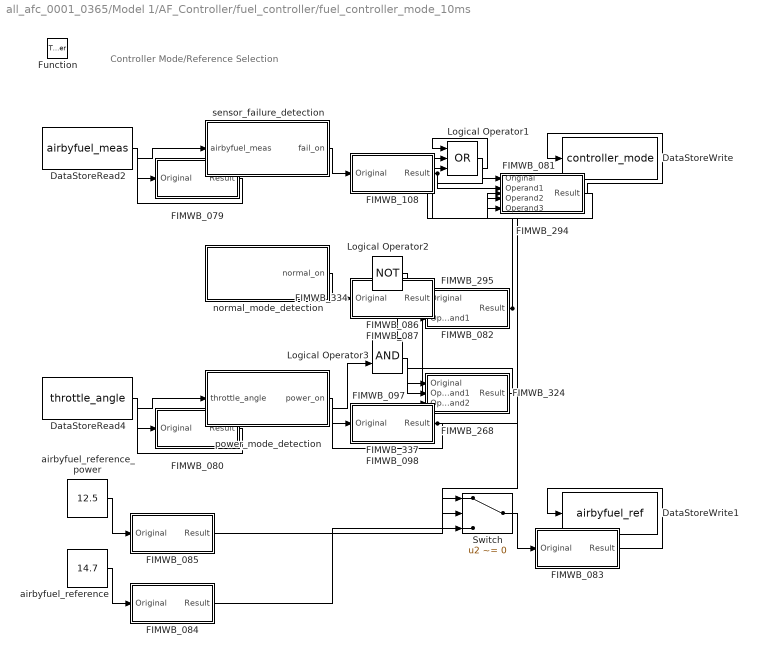
== system all_afc_0001_0365/Model 1/AF_Controller/fuel_controller/fuel_controller_mode_10ms ==
  note: Controller Mode/Reference Selection
  Function : TriggerPort  VariantControl=(inherit)
  DataStoreRead2 : DataStoreRead  DataStoreName=airbyfuel_meas  IndexOptions=Index vector (dialog)  Indices=1  OutputSizes=1
  DataStoreRead4 : DataStoreRead  DataStoreName=throttle_angle  IndexOptions=Index vector (dialog)  Indices=1  OutputSizes=1
  DataStoreWrite : DataStoreWrite  DataStoreName=controller_mode  IndexOptions=Index vector (dialog)  Indices=1  OutputSizes=1
      settings: AttributesFormatString=1: Feedforward\n0: Feedforward + Feedback
  DataStoreWrite1 : DataStoreWrite  DataStoreName=airbyfuel_ref  IndexOptions=Index vector (dialog)  Indices=1  OutputSizes=1
  FIMWB_079 : Subsystem  Tag=fimwb.fault.79
  FIMWB_080 : Subsystem  Tag=fimwb.fault.80
  FIMWB_081 : Subsystem  Tag=fimwb.fault.81
  FIMWB_082 : Subsystem  Tag=fimwb.fault.82
  FIMWB_083 : Subsystem  Tag=fimwb.fault.83
  FIMWB_084 : Subsystem  Tag=fimwb.fault.84
  FIMWB_085 : Subsystem  Tag=fimwb.fault.85
  FIMWB_086 : Subsystem  Tag=fimwb.fault.86
  FIMWB_087 : Subsystem  Tag=fimwb.fault.87
  FIMWB_097 : Subsystem  Tag=fimwb.fault.97
  FIMWB_098 : Subsystem  Tag=fimwb.fault.98
  FIMWB_108 : Subsystem  Tag=fimwb.fault.108
  FIMWB_268 : Subsystem  Tag=fimwb.fault.268
  FIMWB_294 : Subsystem  Tag=fimwb.fault.294
  FIMWB_295 : Subsystem  Tag=fimwb.fault.295
  FIMWB_324 : Subsystem  Tag=fimwb.fault.324
  FIMWB_334 : Subsystem  Tag=fimwb.fault.334
  FIMWB_337 : Subsystem  Tag=fimwb.fault.337
  Logical Operator1 : Logic  Operator=OR  Inputs=3  AllPortsSameDT=off  OutDataTypeStr=boolean
  Logical Operator2 : Logic  Operator=NOT  AllPortsSameDT=off  OutDataTypeStr=boolean
  Logical Operator3 : Logic  AllPortsSameDT=off  OutDataTypeStr=boolean
  Switch : Switch  Criteria=u2 ~= 0  SaturateOnIntegerOverflow=off  InputSameDT=off
  airbyfuel_reference : Constant  Value=14.7  OutDataTypeStr=single  SampleTime=-1
  airbyfuel_reference_power : Constant  Value=12.5  OutDataTypeStr=single  SampleTime=-1
  normal_mode_detection : Subsystem  TreatAsAtomicUnit=on
      settings: AttributesFormatString=0: Feedforward\n1: Feedforward + Feedback
  power_mode_detection : Subsystem  TreatAsAtomicUnit=on
      settings: AttributesFormatString=1: Feedforward\n0: Feedforward + Feedback
  sensor_failure_detection : Subsystem  TreatAsAtomicUnit=on
      settings: AttributesFormatString=1: Feedforward\n0: Feedforward + Feedback
  wires:
  Logical Operator1/1 -> FIMWB_294/1(Original)
  Logical Operator2/1 -> FIMWB_295/1(Original)
  Logical Operator3/1 -> FIMWB_324/1(Original)
  normal_mode_detection/1(normal_on) -> FIMWB_334/1(Original)
  FIMWB_334/1(Result) -> FIMWB_086/1(Original), FIMWB_087/1(Original)
  power_mode_detection/1(power_on) -> FIMWB_337/1(Original)
  FIMWB_337/1(Result) -> FIMWB_097/1(Original), FIMWB_098/1(Original)
  DataStoreRead2/1 -> FIMWB_079/1(Original)
  FIMWB_079/1(Result) -> sensor_failure_detection/1(airbyfuel_meas)
  DataStoreRead4/1 -> FIMWB_080/1(Original)
  FIMWB_080/1(Result) -> power_mode_detection/1(throttle_angle)
  FIMWB_294/1(Result) -> FIMWB_081/1(Original)
  FIMWB_081/1(Result) -> DataStoreWrite/1
  FIMWB_295/1(Result) -> FIMWB_082/1(Original)
  FIMWB_082/1(Result) -> Logical Operator1/2, FIMWB_294/3(Operand2)
  Switch/1 -> FIMWB_083/1(Original)
  FIMWB_083/1(Result) -> DataStoreWrite1/1
  airbyfuel_reference/1 -> FIMWB_084/1(Original)
  FIMWB_084/1(Result) -> Switch/3
  airbyfuel_reference_power/1 -> FIMWB_085/1(Original)
  FIMWB_085/1(Result) -> Switch/1
  FIMWB_086/1(Result) -> Logical Operator2/1, FIMWB_295/2(Operand1)
  FIMWB_087/1(Result) -> Logical Operator3/1, FIMWB_324/2(Operand1)
  FIMWB_097/1(Result) -> Logical Operator1/3, FIMWB_294/4(Operand3)
  FIMWB_098/1(Result) -> Logical Operator3/2, FIMWB_324/3(Operand2)
  sensor_failure_detection/1(fail_on) -> FIMWB_108/1(Original)
  FIMWB_108/1(Result) -> Logical Operator1/1, FIMWB_294/2(Operand1)
  FIMWB_324/1(Result) -> FIMWB_268/1(Original)
  FIMWB_268/1(Result) -> Switch/2

== system all_afc_0001_0365/Model 1/AF_Controller/fuel_controller/fuel_controller_pwon ==
  Function : TriggerPort  VariantControl=(inherit)
  Constant1 : Constant  OutDataTypeStr=single  SampleTime=-1
  Constant2 : Constant  Value=0.1726  OutDataTypeStr=single  SampleTime=-1
  Constant3 : Constant  Value=14.7  OutDataTypeStr=single  SampleTime=-1
  Data Type Conversion : DataTypeConversion  OutDataTypeStr=boolean  SaturateOnIntegerOverflow=off  RndMeth=Floor
  DataStoreWrite : DataStoreWrite  DataStoreName=commanded_fuel  IndexOptions=Index vector (dialog)  Indices=1  OutputSizes=1
  DataStoreWrite1 : DataStoreWrite  DataStoreName=controller_mode  IndexOptions=Index vector (dialog)  Indices=1  OutputSizes=1
  DataStoreWrite2 : DataStoreWrite  DataStoreName=airbyfuel_ref  IndexOptions=Index vector (dialog)  Indices=1  OutputSizes=1
  FIMWB_115 : Subsystem  Tag=fimwb.fault.115
  FIMWB_116 : Subsystem  Tag=fimwb.fault.116
  FIMWB_117 : Subsystem  Tag=fimwb.fault.117
  FIMWB_118 : Subsystem  Tag=fimwb.fault.118
  wires:
  Constant1/1 -> FIMWB_115/1(Original)
  FIMWB_115/1(Result) -> Data Type Conversion/1
  Constant2/1 -> FIMWB_116/1(Original)
  FIMWB_116/1(Result) -> DataStoreWrite/1
  Constant3/1 -> FIMWB_117/1(Original)
  FIMWB_117/1(Result) -> DataStoreWrite2/1
  Data Type Conversion/1 -> FIMWB_118/1(Original)
  FIMWB_118/1(Result) -> DataStoreWrite1/1

== system all_afc_0001_0365/Model 1/Cylinder and Exhaust/A//F_sensor/FIMWB_133 ==
  Original : Inport
  Result : Outport
  wires:
  Original/1 -> Result/1

== system all_afc_0001_0365/Model 1/Cylinder and Exhaust/A//F_sensor/FIMWB_134 ==
  Original : Inport
  Result : Outport
  wires:
  Original/1 -> Result/1

== system all_afc_0001_0365/Model 1/Cylinder and Exhaust/A//F_sensor/FIMWB_135 ==
  Original : Inport
  Result : Outport
  wires:
  Original/1 -> Result/1

== system all_afc_0001_0365/Model 1/Cylinder and Exhaust/A//F_sensor/Filter ==
  In : Inport
  FIMWB_136 : Subsystem  Tag=fimwb.fault.136
  FIMWB_137 : Subsystem  Tag=fimwb.fault.137
  FIMWB_138 : Subsystem  Tag=fimwb.fault.138
  FIMWB_139 : Subsystem  Tag=fimwb.fault.139
  FIMWB_140 : Subsystem  Tag=fimwb.fault.140
  FIMWB_303 : Subsystem  Tag=fimwb.fault.303
  FIMWB_345 : Subsystem  Tag=fimwb.fault.345
  Gain : Gain  Gain=50
  Integrator : Integrator  InitialCondition=14.7
  Sum : Sum  Inputs=|+-
  Out : Outport  VectorParamsAs1DForOutWhenUnconnected=off
  wires:
  Sum/1 -> FIMWB_303/1(Original)
  Integrator/1 -> FIMWB_345/1(Original)
  FIMWB_345/1(Result) -> FIMWB_138/1(Original), FIMWB_139/1(Original)
  In/1 -> FIMWB_136/1(Original)
  FIMWB_136/1(Result) -> Sum/1, FIMWB_303/2(Operand1)
  Gain/1 -> FIMWB_137/1(Original)
  FIMWB_137/1(Result) -> Integrator/1
  FIMWB_138/1(Result) -> Sum/2, FIMWB_303/3(Operand2)
  FIMWB_139/1(Result) -> Out/1
  FIMWB_303/1(Result) -> FIMWB_140/1(Original)
  FIMWB_140/1(Result) -> Gain/1

== system all_afc_0001_0365/Model 1/Cylinder and Exhaust/Filter/FIMWB_144 ==
  Original : Inport
  Result : Outport
  wires:
  Original/1 -> Result/1

== system all_afc_0001_0365/Model 1/Cylinder and Exhaust/Filter/FIMWB_145 ==
  Original : Inport
  Result : Outport
  wires:
  Original/1 -> Result/1

== system all_afc_0001_0365/Model 1/Cylinder and Exhaust/Filter/FIMWB_146 ==
  Original : Inport
  Result : Outport
  wires:
  Original/1 -> Result/1

== system all_afc_0001_0365/Model 1/Cylinder and Exhaust/Filter/FIMWB_147 ==
  Original : Inport
  Result : Outport
  wires:
  Original/1 -> Result/1

== system all_afc_0001_0365/Model 1/Cylinder and Exhaust/Filter/FIMWB_148 ==
  Original : Inport
  Result : Outport
  wires:
  Original/1 -> Result/1

== system all_afc_0001_0365/Model 1/Cylinder and Exhaust/Filter/FIMWB_305 ==
  Original : Inport
  Operand1 : Inport  Port=2
  Operand2 : Inport  Port=3
  Unused2 : Terminator
  Unused3 : Terminator
  Result : Outport
  wires:
  Original/1 -> Result/1
  Operand1/1 -> Unused2/1
  Operand2/1 -> Unused3/1

== system all_afc_0001_0365/Model 1/Cylinder and Exhaust/Filter/FIMWB_346 ==
  Original : Inport
  Result : Outport
  wires:
  Original/1 -> Result/1

== system all_afc_0001_0365/V&V stub system/Calcuate Error/RMS error/FIMWB_248 ==
  Original : Inport
  Result : Outport
  wires:
  Original/1 -> Result/1

== system all_afc_0001_0365/V&V stub system/Calcuate Error/RMS error/FIMWB_249 ==
  Original : Inport
  Result : Outport
  wires:
  Original/1 -> Result/1

== system all_afc_0001_0365/V&V stub system/Calcuate Error/RMS error/FIMWB_250 ==
  Original : Inport
  Result : Outport
  wires:
  Original/1 -> Result/1

== system all_afc_0001_0365/V&V stub system/Calcuate Error/RMS error/FIMWB_251 ==
  Original : Inport
  Result : Outport
  wires:
  Original/1 -> Result/1

== system all_afc_0001_0365/V&V stub system/Calcuate Error/RMS error/FIMWB_252 ==
  Original : Inport
  Result : Outport
  wires:
  Original/1 -> Result/1

== system all_afc_0001_0365/V&V stub system/Calcuate Error/RMS error/FIMWB_253 ==
  Original : Inport
  Result : Outport
  wires:
  Original/1 -> Result/1

== system all_afc_0001_0365/V&V stub system/Calcuate Error/RMS error/FIMWB_254 ==
  Original : Inport
  Result : Outport
  wires:
  Original/1 -> Result/1

== system all_afc_0001_0365/V&V stub system/Calcuate Error/RMS error/FIMWB_266 ==
  Original : Inport
  Result : Outport
  wires:
  Original/1 -> Result/1

== system all_afc_0001_0365/V&V stub system/Calcuate Error/RMS error/FIMWB_267 ==
  Original : Inport
  Result : Outport
  wires:
  Original/1 -> Result/1

== system all_afc_0001_0365/V&V stub system/Calcuate Error/RMS error/FIMWB_270 ==
  Original : Inport
  Result : Outport
  wires:
  Original/1 -> Result/1

== system all_afc_0001_0365/V&V stub system/Calcuate Error/RMS error/FIMWB_319 ==
  Original : Inport
  Operand1 : Inport  Port=2
  Operand2 : Inport  Port=3
  Unused2 : Terminator
  Unused3 : Terminator
  Result : Outport
  wires:
  Original/1 -> Result/1
  Operand1/1 -> Unused2/1
  Operand2/1 -> Unused3/1

== system all_afc_0001_0365/V&V stub system/Calcuate Error/RMS error/FIMWB_320 ==
  Original : Inport
  Operand1 : Inport  Port=2
  Operand2 : Inport  Port=3
  Unused2 : Terminator
  Unused3 : Terminator
  Result : Outport
  wires:
  Original/1 -> Result/1
  Operand1/1 -> Unused2/1
  Operand2/1 -> Unused3/1

== system all_afc_0001_0365/V&V stub system/Calcuate Error/RMS error/FIMWB_323 ==
  Original : Inport
  Operand1 : Inport  Port=2
  Operand2 : Inport  Port=3
  Unused2 : Terminator
  Unused3 : Terminator
  Result : Outport
  wires:
  Original/1 -> Result/1
  Operand1/1 -> Unused2/1
  Operand2/1 -> Unused3/1

== system all_afc_0001_0365/V&V stub system/Calcuate Error/over(under)shoot/FIMWB_256 ==
  Original : Inport
  Result : Outport
  wires:
  Original/1 -> Result/1

== system all_afc_0001_0365/V&V stub system/Calcuate Error/over(under)shoot/FIMWB_257 ==
  Original : Inport
  Result : Outport
  wires:
  Original/1 -> Result/1

== system all_afc_0001_0365/V&V stub system/Calcuate Error/over(under)shoot/FIMWB_258 ==
  Original : Inport
  Result : Outport
  wires:
  Original/1 -> Result/1

== system all_afc_0001_0365/V&V stub system/Calcuate Error/over(under)shoot/FIMWB_259 ==
  Original : Inport
  Result : Outport
  wires:
  Original/1 -> Result/1

== system all_afc_0001_0365/V&V stub system/Calcuate Error/over(under)shoot/FIMWB_271 ==
  Original : Inport
  Result : Outport
  wires:
  Original/1 -> Result/1

== system all_afc_0001_0365/V&V stub system/Calcuate Error/over(under)shoot/FIMWB_321 ==
  Original : Inport
  Operand1 : Inport  Port=2
  Operand2 : Inport  Port=3
  Unused2 : Terminator
  Unused3 : Terminator
  Result : Outport
  wires:
  Original/1 -> Result/1
  Operand1/1 -> Unused2/1
  Operand2/1 -> Unused3/1

== system all_afc_0001_0365/V&V stub system/Calcuate Error/over(under)shoot/FIMWB_322 ==
  Original : Inport
  Operand1 : Inport  Port=2
  Operand2 : Inport  Port=3
  Unused2 : Terminator
  Unused3 : Terminator
  Result : Outport
  wires:
  Original/1 -> Result/1
  Operand1/1 -> Unused2/1
  Operand2/1 -> Unused3/1

== system all_afc_0001_0365/Model 1/AF_Controller/fuel_controller/fuel_controller_10ms/FIMWB_025 ==
  Original : Inport
  Result : Outport
  wires:
  Original/1 -> Result/1

== system all_afc_0001_0365/Model 1/AF_Controller/fuel_controller/fuel_controller_10ms/FIMWB_026 ==
  Original : Inport
  Result : Outport
  wires:
  Original/1 -> Result/1

== system all_afc_0001_0365/Model 1/AF_Controller/fuel_controller/fuel_controller_10ms/FIMWB_027 ==
  Original : Inport
  Result : Outport
  wires:
  Original/1 -> Result/1

== system all_afc_0001_0365/Model 1/AF_Controller/fuel_controller/fuel_controller_10ms/FIMWB_028 ==
  Original : Inport
  Result : Outport
  wires:
  Original/1 -> Result/1

== system all_afc_0001_0365/Model 1/AF_Controller/fuel_controller/fuel_controller_10ms/FIMWB_029 ==
  Original : Inport
  Result : Outport
  wires:
  Original/1 -> Result/1

== system all_afc_0001_0365/Model 1/AF_Controller/fuel_controller/fuel_controller_10ms/FIMWB_030 ==
  Original : Inport
  Result : Outport
  wires:
  Original/1 -> Result/1

== system all_afc_0001_0365/Model 1/AF_Controller/fuel_controller/fuel_controller_10ms/FIMWB_031 ==
  Original : Inport
  Result : Outport
  wires:
  Original/1 -> Result/1

== system all_afc_0001_0365/Model 1/AF_Controller/fuel_controller/fuel_controller_10ms/FIMWB_032 ==
  Original : Inport
  Result : Outport
  wires:
  Original/1 -> Result/1

== system all_afc_0001_0365/Model 1/AF_Controller/fuel_controller/fuel_controller_10ms/FIMWB_033 ==
  Original : Inport
  Result : Outport
  wires:
  Original/1 -> Result/1

== system all_afc_0001_0365/Model 1/AF_Controller/fuel_controller/fuel_controller_10ms/FIMWB_034 ==
  Original : Inport
  Result : Outport
  wires:
  Original/1 -> Result/1

== system all_afc_0001_0365/Model 1/AF_Controller/fuel_controller/fuel_controller_10ms/FIMWB_035 ==
  Original : Inport
  Result : Outport
  wires:
  Original/1 -> Result/1

== system all_afc_0001_0365/Model 1/AF_Controller/fuel_controller/fuel_controller_10ms/FIMWB_036 ==
  Original : Inport
  Result : Outport
  wires:
  Original/1 -> Result/1

== system all_afc_0001_0365/Model 1/AF_Controller/fuel_controller/fuel_controller_10ms/FIMWB_037 ==
  Original : Inport
  Result : Outport
  wires:
  Original/1 -> Result/1

== system all_afc_0001_0365/Model 1/AF_Controller/fuel_controller/fuel_controller_10ms/FIMWB_062 ==
  Original : Inport
  Result : Outport
  wires:
  Original/1 -> Result/1

== system all_afc_0001_0365/Model 1/AF_Controller/fuel_controller/fuel_controller_10ms/FIMWB_063 ==
  Original : Inport
  Result : Outport
  wires:
  Original/1 -> Result/1

== system all_afc_0001_0365/Model 1/AF_Controller/fuel_controller/fuel_controller_10ms/FIMWB_074 ==
  Original : Inport
  Result : Outport
  wires:
  Original/1 -> Result/1

== system all_afc_0001_0365/Model 1/AF_Controller/fuel_controller/fuel_controller_10ms/FIMWB_078 ==
  Original : Inport
  Result : Outport
  wires:
  Original/1 -> Result/1

== system all_afc_0001_0365/Model 1/AF_Controller/fuel_controller/fuel_controller_10ms/FIMWB_281 ==
  Original : Inport
  Operand1 : Inport  Port=2
  Operand2 : Inport  Port=3
  Unused2 : Terminator
  Unused3 : Terminator
  Result : Outport
  wires:
  Original/1 -> Result/1
  Operand1/1 -> Unused2/1
  Operand2/1 -> Unused3/1

== system all_afc_0001_0365/Model 1/AF_Controller/fuel_controller/fuel_controller_10ms/FIMWB_282 ==
  Original : Inport
  Operand1 : Inport  Port=2
  Operand2 : Inport  Port=3
  Unused2 : Terminator
  Unused3 : Terminator
  Result : Outport
  wires:
  Original/1 -> Result/1
  Operand1/1 -> Unused2/1
  Operand2/1 -> Unused3/1

== system all_afc_0001_0365/Model 1/AF_Controller/fuel_controller/fuel_controller_10ms/FIMWB_328 ==
  Original : Inport
  Result : Outport
  wires:
  Original/1 -> Result/1

== system all_afc_0001_0365/Model 1/AF_Controller/fuel_controller/fuel_controller_10ms/FIMWB_329 ==
  Original : Inport
  Result : Outport
  wires:
  Original/1 -> Result/1
